simulink model "arducopter"  (R2021a)
settings: Solver=FixedStepAuto  StartTime=0.0  StopTime=simIn.param.timeEnd  FixedStep=simIn.param.dt  RelTol=1e-3
undefined symbols (not defined in the file or in its folder): DiscIntNeverNeededParam, sim, simIn
libraries: simulink x35, slident x4, vrlib x1
(part 9 of 9)

== matlab function arducopter/radioIn to controlIn/MATLAB Function ==
  data: rcIn input; angleIn output; deadZone input; radioMin input; radioMax input; trim input; reversed input; highIn input
function angleIn = pwm_to_angle_dz(rcIn, deadZone, radioMin, radioMax, trim, reversed, highIn)
% Computes a angle in centidegree value from the current radio_in value
% using the specified dead_zone and trim
% Code based on RC_Channel::pwm_to_angle_dz() and RC_Channel::pwm_to_angle_dz_trim()

radioTrimHigh = trim + deadZone;
radioTrimLow = trim - deadZone;

if reversed
    reverseMul = -1;
else
    reverseMul = 1;
end

% Dont allow out of range values
rcIn = max(min(rcIn, radioMax), radioMin);

if rcIn > radioTrimHigh && radioMax ~= radioTrimHigh
    angleIn = reverseMul * highIn * (rcIn - radioTrimHigh) / (radioMax  - radioTrimHigh);
elseif rcIn < radioTrimLow && radioTrimLow ~= radioMin
    angleIn = reverseMul * highIn * (rcIn - radioTrimLow) / (radioTrimLow - radioMin);
else
    angleIn = single(0);
end

== matlab function arducopter/radioIn to controlIn/MATLAB Function1 ==
  data: radioIn input; out output; deadZone input; radioTrim input; radioMin input; radioMax input; reversed input
function out = norm_input_dz(radioIn, deadZone, radioTrim, radioMin, radioMax, reversed)
% Code based on RC_Channel::norm_input_dz()
dzMin = radioTrim - deadZone;
dzMax = radioTrim + deadZone;

if reversed
    revMult = -1;
else
    revMult = 1;
end

if radioIn < dzMin && dzMin > radioMin
    out = revMult * (radioIn - dzMin) / (dzMin - radioMin);
elseif radioIn > dzMax && radioMax > dzMax
    out = revMult * (radioIn - dzMax) / (radioMax - dzMax);
else
    out = single(0);
end

out = min(max(out, single(-1)), single(1));

== matlab function arducopter/Rate Controller/PID Pitch Rate/Slew Limiter/Calculate Dmod1 ==
  data: slew_rate input; Dmod output single; sr_max input; sr_tau input; dt input; time input; pos_event_idx data_store_memory; pos_event_stored data_store_memory; pos_event_ms data_store_memory; neg_event_idx data_store_memory; neg_event_stored data_store_memory; neg_event_ms data_store_memory; modifier_slew_rate data_store_memory; output_slew_rate data_store_memory; max_neg_slew_event_ms data_store_memory; max_pos_slew_event_ms data_store_memory; max_neg_slew_rate data_store_memory; max_pos_slew_rate data_store_memory
function Dmod   = fcn(slew_rate, sr_max, sr_tau, dt, time)
% Code is based on SlewLimiter::modifier() in SlewLimiter.cpp. 

% Define global variables, so that quanitities do not have to be fed back
% to the function
global pos_event_stored;
global pos_event_idx;
global pos_event_ms;
global max_pos_slew_rate;
global max_pos_slew_event_ms;
global neg_event_stored;
global neg_event_idx;
global neg_event_ms;
global max_neg_slew_rate;
global max_neg_slew_event_ms;
global modifier_slew_rate;
global output_slew_rate;

% Definition of constants as done in SlewLimiter.h
N_EVENTS = uint32(3); % Number of positive and negative consecutive slew rate exceedance events recorded. Set to 3 because of 1-based indexing.
WINDOW_MS = uint32(300); % Time in ms required for half a cycle of the slowest oscillation frequency expected
MODIFIER_GAIN = 1.5; % Ratio of modifier reduction to slew rate exceedance

% Check if slew limiter is activated
if(sr_max <= 0)
   Dmod = single(1.0);
end

now_ms = uint32(time);
decay_alpha = min(dt, sr_tau) / sr_tau;

%% Save exceedance events in event time vector
% Store a series of positive slew rate exceedance events
if (~pos_event_stored && slew_rate > sr_max)
    if (pos_event_idx >= N_EVENTS)
        pos_event_idx(:) = 1;
    end
    pos_event_ms(pos_event_idx) = now_ms;
    pos_event_idx(:) = pos_event_idx + 1;
    pos_event_stored = true;
    neg_event_stored = false;
end

% Store a series of negative slew rate exceedance events
if (~neg_event_stored && slew_rate < -sr_max)
    if (neg_event_idx >= N_EVENTS)
        neg_event_idx(:) = 1;
    end
    neg_event_ms(neg_event_idx) = now_ms;
    neg_event_idx(:) = neg_event_idx + 1;
    pos_event_stored = false;
    neg_event_stored = true;
end

% Find oldest event time
oldest_ms = now_ms;
for i=1:N_EVENTS-1
   if (pos_event_ms(i) < oldest_ms)
       oldest_ms = pos_event_ms(i);
   end
   if (neg_event_ms(i) < oldest_ms)
       oldest_ms = neg_event_ms(i);
   end
end

%% Calculate maximum slew rate
% Save new maximum slew rates, if oldest maximum is exceeded
% OR decay the peak slew rates (pos. and neg.) if they are outside the
% observed time window
if (slew_rate > max_pos_slew_rate)
    max_pos_slew_rate(:) = min(slew_rate, 10 * sr_max);
    max_pos_slew_event_ms = now_ms;
elseif (now_ms - max_pos_slew_event_ms > WINDOW_MS)
    max_pos_slew_rate = max_pos_slew_rate * (1.0 - decay_alpha);
end

if (slew_rate < -max_neg_slew_rate)
    max_neg_slew_rate(:) = min(-slew_rate, 10 * sr_max);
    max_neg_slew_event_ms = now_ms;
elseif (now_ms - max_neg_slew_event_ms > WINDOW_MS)
    max_neg_slew_rate = max_neg_slew_rate * (1.0 - decay_alpha);
end

% Calculate the averaged maximum slew rate
raw_slew_rate = 0.5 * (max_pos_slew_rate + max_neg_slew_rate);

% When the oldest exceedance event falls outside of the window required for
% the number of exceedance events, apply a further reduction to the maximum
% slew rate. This prevents unwanted gain reductions caused by spikes in the
% demanded angular rates due to changed control modes or similar causes.
modifier_input = raw_slew_rate;
if(now_ms - oldest_ms > N_EVENTS * WINDOW_MS) % no incrementation of N_EVENTS because of 1 based indexing
   oldest_time_from_window = single(0.001) * single(now_ms - oldest_ms - N_EVENTS * WINDOW_MS); 
   modifier_input = modifier_input * single(exp(-oldest_time_from_window / sr_tau));
end

%% Calculation of modifier and output slew rate

% Apply filter to slew rate in order to reduce effects of large setpoint
% changes
attack_alpha = min(2.0 * decay_alpha, 1.0);

modifier_slew_rate = modifier_slew_rate + (modifier_input - modifier_slew_rate) * attack_alpha;
modifier_slew_rate = min(modifier_slew_rate, modifier_input);

output_slew_rate = output_slew_rate + (raw_slew_rate - output_slew_rate) * attack_alpha;
output_slew_rate = min(raw_slew_rate, output_slew_rate);

% Calculate modifier. Only has an impact if sr_max is exceeded by averaged
% slew rate.
if(modifier_slew_rate > sr_max)
    Dmod(:) = sr_max / (sr_max + MODIFIER_GAIN * (modifier_slew_rate - sr_max));
else
    Dmod(:) = 1.0;
end

== matlab function arducopter/radioIn to controlIn/MATLAB Function3 ==
  data: rcIn input; angleIn output; deadZone input; radioMin input; radioMax input; trim input; reversed input; highIn input
function angleIn = pwm_to_angle_dz(rcIn, deadZone, radioMin, radioMax, trim, reversed, highIn)
% Computes a angle in centidegree value from the current radio_in value
% using the specified dead_zone and trim
% Code based on RC_Channel::pwm_to_angle_dz() and RC_Channel::pwm_to_angle_dz_trim()

radioTrimHigh = trim + deadZone;
radioTrimLow = trim - deadZone;

if reversed
    reverseMul = -1;
else
    reverseMul = 1;
end

% Dont allow out of range values
rcIn = max(min(rcIn, radioMax), radioMin);

if rcIn > radioTrimHigh && radioMax ~= radioTrimHigh
    angleIn = reverseMul * highIn * (rcIn - radioTrimHigh) / (radioMax  - radioTrimHigh);
elseif rcIn < radioTrimLow && radioTrimLow ~= radioMin
    angleIn = reverseMul * highIn * (rcIn - radioTrimLow) / (radioTrimLow - radioMin);
else
    angleIn = single(0);
end

== matlab function arducopter/Throttle/Throttle Calculations/Lowpass Filter/Lowpass Filter with reset ==
  data: in input; out output single; cutoff_freq input; loop_rate input; lastSamp input
function out  = lowpass(in, cutoff_freq, loop_rate, lastSamp)
%% The code is based on the apply(sample, cutoff_freq, dt) function in LowPassFilter.cpp.
dt = 1 / loop_rate;

% Check if filter is supposed to be filtering
if (cutoff_freq <=0 || dt <= 0)
    out = in;
else
    % Calculate time constant and alpha value
    T = 1 / (2 * pi * cutoff_freq);
    alpha = dt / (dt + T);
    alpha = max( min( alpha, 1.0), 0.0);
    
    % Output calculation
    out = lastSamp + (in - lastSamp) * alpha;
end

%% Code is based on AP_MotorsMulticopter::update_throttle_filter(), in AP_MotorsMulticopter.cpp.
% If the output surpases the limits [0,1], the filter is reset (according
% to the reset() function in LowPassFilter.cpp.)
if (out < single(0.0))
   out = single(0.0); 

elseif (out > 1.0)
    out = single(1.0);
end

== matlab function arducopter/Rate Controller/PID Pitch Rate/Slew Limiter/Lowpass Filter1 ==
  data: in input; out output single; cutoff_freq input; loop_rate input; out_last input
function out  = fcn(in, cutoff_freq, loop_rate, out_last)
% The code is based on the apply(sample, cutoff_freq, dt) function in
% LowPassFilter.cpp
dt = 1 / loop_rate;

% Check if filter is supposed to be filtering
if (cutoff_freq <=0 || dt <= 0)
    out = in;
    return;
end

% Calculate time constant and alpha value
T = 1 / (2 * pi * cutoff_freq);
alpha = dt / (dt + T);
alpha = max( min( alpha, 1.0), 0.0);

% Output calculation
out = out_last + (in - out_last) * alpha;

== matlab function arducopter/Attitude Controller/input_euler_angle_roll_pitch_euler_rate_yaw()/reset yaw targets/MATLAB Function5 ==
  data: vec input; q output
function q = fromAxisAngle(vec)
% Create a quaternion from its axis-angle representation. Just the rotation
% vector is given as input.
% Based on QuaternionT<T>::from_axis_angle(Vector3<T>)

q = zeros(4,1);
angle = single(sqrt(vec(1)^2 + vec(2)^2 + vec(3)^2));

if angle == 0
    q(1) = single(1);
    q(2) = single(0);
    q(3) = single(0);
    q(4) = single(0);
else
    axis = vec ./ angle;
    % The following lines are based on QuaternionT<T>::from_axis_angle(const Vector3<T> &axis, T theta)
    if angle == 0
        q(1) = single(1);
        q(2) = single(0);
        q(3) = single(0);
        q(4) = single(0);
    else
        st2 = single(sin(0.5*angle));
        q(1) = single(cos(0.5*angle));
        q(2) = axis(1) * st2;
        q(3) = axis(2) * st2;
        q(4) = axis(3) * st2;
    end
end

== matlab function arducopter/radioIn to controlIn/MATLAB Function2 ==
  data: rcIn input; ctrlIn output; deadZone input; radioMin input; radioMax input; reversed input; highIn input
function ctrlIn = pwm_to_range_dz(rcIn, deadZone, radioMin, radioMax, reversed, highIn)
% Converts a pwm value to a value in the configured range
% Code based on RC_Channel::pwm_to_range_dz()

rcIn = max(min(rcIn, radioMax), radioMin);

if reversed
    rcIn = radioMax - (rcIn - radioMin);
end

radioTrimLow = radioMin + deadZone;

if rcIn > radioTrimLow
    ctrlIn = highIn * (rcIn - radioTrimLow) / (radioMax - radioTrimLow);
else
    ctrlIn = single(0);
end

== matlab function arducopter/Position Controller/calc des climb rate/MATLAB Function ==
  data: ctrlIn input; climbRateDes output; deadZoneThr input; deadZoneRC input; radioMin input; radioMax input; reversed input; highIn input; maxSpeedDn input; maxSpeedUp input
function climbRateDes = get_pilot_desired_climb_rate(ctrlIn, deadZoneThr, deadZoneRC, radioMin, radioMax, reversed, highIn, maxSpeedDn, maxSpeedUp)
% Calculation of the desired climb rate based on the pilot's throttle input
% Based on Copter::get_pilot_desired_climb_rate()

% Ensure a reasonable throttle value
ctrlIn = min(max(ctrlIn, 0), 1000);

% Ensure a reasonable deadzone
thrDz = min(max(deadZoneThr, 0), 400);

% Calculation of mid_stick based on Copter::get_throttle_mid()
rIn = (radioMin + radioMax) / 2;
if reversed
    rIn = radioMax - (rIn - radioMin);
end
radioTrimLow = radioMin + deadZoneRC;
midStick = highIn * (rIn - radioTrimLow) / (radioMax - radioTrimLow);

deadbandTop = midStick + thrDz;
deadbandBottom = midStick - thrDz;

% Check throttle is above, below or in the deadband
if ctrlIn < deadbandBottom
    % Below deadband
    % Get maximum down speed that can be demanded by pilot. If zero, the
    % maximum up speed is used according to get_pilot_speed_dn()
    if maxSpeedDn == 0
        maxSpeedDn = abs(maxSpeedUp);
    end
    climbRateDes = maxSpeedDn * (ctrlIn - deadbandBottom) / deadbandBottom;
elseif ctrlIn > deadbandTop
    % Above deadband
    climbRateDes = maxSpeedUp * (ctrlIn - deadbandTop) / (1000 - deadbandTop);
else
    % In the deadband
    climbRateDes = single(0); 
end

== matlab function arducopter/Position Controller/set_pos_target_z_from_climb_rate()/input_vel_accel_z/MATLAB Function ==
  data: overspeedGain output; velMaxUp input; velMaxDn input; velDes input; overspeedGainDefault input
function overspeedGain = calcOverspeedGain(velMaxUp, velMaxDn, velDes, overspeedGainDefault)
% Calculate increased maximum acceleration and jerk if over speed condition
% is detected
% Code based on AC_PosControl::calculate_overspeed_gain()
overspeedGain = single(1);
if velDes < velMaxDn && velMaxDn ~= 0
    overspeedGain = overspeedGainDefault * velDes / velMaxDn;
end
if velDes > velMaxUp && velMaxUp ~= 0
    overspeedGain = overspeedGainDefault * velDes / velMaxUp;
end
